simulink library "Lib_Piccolo"  (R2018b)
settings: Solver=VariableStepAuto  StartTime=0.0  StopTime=10.0  RelTol=1e-3
values from neighbouring files (symbols this model uses):
  AccelErrInt2Brakes = 0.15    [SimulationControlConfig16P.m]    (also in SimulationControlConfig16P_LEGACY.m; SimulationControlConfigTAILLESS.m = 0.2; SimulationControlConfigUTAIL.m = 0.2)
  AileronMax = 25    [SimulationControlConfig16P.m]    (also in SimulationControlConfig16P_LEGACY.m; SimulationControlConfigTAILLESS.m; SimulationControlConfigUTAIL.m)
  AileronPower = 0.00268    [SimulationControlConfig16P.m]    (also in SimulationControlConfig16P_LEGACY.m; SimulationControlConfigTAILLESS.m; SimulationControlConfigUTAIL.m)
  AileronSurfaceMax = 45    [SimulationControlConfig16P.m]    (also in SimulationControlConfig16P_LEGACY.m)
  AileronTrim = 0    [SimulationControlConfig16P.m]    (also in SimulationControlConfig16P_LEGACY.m; SimulationControlConfigTAILLESS.m; SimulationControlConfigUTAIL.m)
  Alt = 1000 + TerrainHeight    [SimulationStateConfig.m]
  AltCruise_m = testPlans(testIndx).terrainElevation * 0.3048 + 200    [SimulationControlConfig16P.m]    (also in SimulationControlConfigTAILLESS.m = 1083; SimulationControlConfigUTAIL.m = testPlans(testIndx).terrainElevation * 0.3048 + 152)
  AltitudeRate2PitchCmdIntegratorInit = 0.1    [SimulationControlPre.m]
  AltMax = 10000    [SimulationControlConfig16P.m]    (also in SimulationControlConfig16P_LEGACY.m; SimulationControlConfigTAILLESS.m; SimulationControlConfigUTAIL.m)
  AltMaxAccel = 1.25    [SimulationControlConfig16P.m]    (also in SimulationControlConfig16P_LEGACY.m = 0.9; SimulationControlConfigTAILLESS.m = 1.7; SimulationControlConfigUTAIL.m = 2)
  AltMin = 0    [SimulationControlConfig16P.m]    (also in SimulationControlConfig16P_LEGACY.m; SimulationControlConfigTAILLESS.m; SimulationControlConfigUTAIL.m)
  AltRateCmd2Pitch = 0.50    (= 0.5)    [SimulationControlConfig16P.m]    (also in SimulationControlConfig16P_LEGACY.m = 0.6; SimulationControlConfigTAILLESS.m = 0.2; SimulationControlConfigUTAIL.m = 0.3)
  AltRateError2Pitch = 0.40    (= 0.4)    [SimulationControlConfig16P.m]    (also in SimulationControlConfig16P_LEGACY.m; SimulationControlConfigTAILLESS.m = 0.55; SimulationControlConfigUTAIL.m = 0.55)
  AltRateErrorInt2Pitch = 0.50    (= 0.5)    [SimulationControlConfig16P.m]    (also in SimulationControlConfig16P_LEGACY.m = 0.45; SimulationControlConfigTAILLESS.m; SimulationControlConfigUTAIL.m = 0.75)
  AltRateLpfCutOff = 3    [SimulationControlConfig16P.m]    (also in SimulationControlConfig16P_LEGACY.m; SimulationControlConfigTAILLESS.m = 2; SimulationControlConfigUTAIL.m = 2)
  AutoNosegear2Rudder = 26    [SimulationControlConfig16P.m]    (also in SimulationControlConfig16P_LEGACY.m; SimulationControlConfigTAILLESS.m = 25.2; SimulationControlConfigUTAIL.m = 14)
  b = 5.54    [SimulationControlConfig16P.m]    (also in SimulationControlConfig16P_LEGACY.m; SimulationControlConfigTAILLESS.m = 2.37; SimulationControlConfigUTAIL.m = 2.37)
  Bank2AileronIntegratorInit = 0    [SimulationControlPre.m]
  BankMax_User = BankMax_User/180*pi    (= 0.523598775598)    [SimulationControlConfig16P.m]    (also in SimulationControlConfig16P_LEGACY.m; SimulationControlConfigTAILLESS.m = 0.610865238198; SimulationControlConfigUTAIL.m = 0.628318530718)
  baseLegFlaps = 20    [SimulationControlConfig16P.m]    (also in SimulationControlConfig16P_LEGACY.m = 0; SimulationControlConfigTAILLESS.m = 15; SimulationControlConfigUTAIL.m = 10)
  C = GeneticOpt.C    [SimulationCostFunction.m]
  c = Sw/b    (= 0.841696750903)    [SimulationControlConfig16P.m]    (also in SimulationControlConfig16P_LEGACY.m; SimulationControlConfigTAILLESS.m = 0.354008438819; SimulationControlConfigUTAIL.m = 0.354008438819)
  cell2WheelFactorMG = 5.98    [SimulationSensorConfig16P_LEGACY.m]
  cell2WheelFactorNG = 1    [SimulationSensorConfig16P_LEGACY.m]
  cellSatMaxMG = 15000    [SimulationSensorConfig16P.m]    (also in SimulationSensorConfig16P_LEGACY.m; SimulationSensorConfigTAILLESS7P.m; SimulationSensorConfigUTAIL7P.m)
  cellSatMaxNG = 1000    [SimulationSensorConfig16P.m]    (also in SimulationSensorConfig16P_LEGACY.m; SimulationSensorConfigTAILLESS7P.m; SimulationSensorConfigUTAIL7P.m)
  cellSatMinMG = -15000    [SimulationSensorConfig16P.m]    (also in SimulationSensorConfig16P_LEGACY.m; SimulationSensorConfigTAILLESS7P.m; SimulationSensorConfigUTAIL7P.m)
  cellSatMinNG = -1000    [SimulationSensorConfig16P.m]    (also in SimulationSensorConfig16P_LEGACY.m; SimulationSensorConfigTAILLESS7P.m; SimulationSensorConfigUTAIL7P.m)
  CL_Limit = CL_Max    (= 0.54)    [SimulationControlConfig16P.m]    (also in SimulationControlConfig16P_LEGACY.m; SimulationControlConfigTAILLESS.m; SimulationControlConfigUTAIL.m = 0.53)
  CL_Max = 0.54    [SimulationControlConfig16P.m]    (also in SimulationControlConfig16P_LEGACY.m; SimulationControlConfigTAILLESS.m; SimulationControlConfigUTAIL.m = 0.53)
  CL_Max_Nom = 0.465    [SimulationControlConfig16P.m]    (also in SimulationControlConfig16P_LEGACY.m; SimulationControlConfigTAILLESS.m = 0.39; SimulationControlConfigUTAIL.m)
  CL_Min = 0    [SimulationControlConfig16P.m]    (also in SimulationControlConfig16P_LEGACY.m; SimulationControlConfigTAILLESS.m; SimulationControlConfigUTAIL.m)
  ClimbMaxFraction = 0.35    [SimulationControlConfig16P.m]    (also in SimulationControlConfig16P_LEGACY.m = 0.24; SimulationControlConfigTAILLESS.m = 0.19; SimulationControlConfigUTAIL.m = 0.21)
  ClimboutMaxBank = 7.0    (= 7)    [SimulationControlConfig16P.m]    (also in SimulationControlConfig16P_LEGACY.m; SimulationControlConfigTAILLESS.m = 5; SimulationControlConfigUTAIL.m)
  ClimboutTimer = 7.0    (= 7)    [SimulationControlConfig16P.m]    (also in SimulationControlConfig16P_LEGACY.m; SimulationControlConfigTAILLESS.m; SimulationControlConfigUTAIL.m)
  dCl_per_dFlap = 0.005581818    [SimulationControlConfig16P.m]    (also in SimulationControlConfig16P_LEGACY.m = 0; SimulationControlConfigTAILLESS.m = 0; SimulationControlConfigUTAIL.m = 0)
  DecelerationCmd = 3.1    [SimulationControlConfig16P.m]    (also in SimulationControlConfig16P_LEGACY.m; SimulationControlConfigTAILLESS.m = 0.1; SimulationControlConfigUTAIL.m = 0.1)
  DeRotateLogicEndTimer = abs((NoseDownLimit_Deg-1)/DeRotateRamp_Dps)    [SimulationControlConfig16P.m]    (also in SimulationControlConfig16P_LEGACY.m; SimulationControlConfigTAILLESS.m; SimulationControlConfigUTAIL.m)
  DeRotateLogicHoldNoseUpTimer = 0.1    [SimulationControlConfig16P.m]    (also in SimulationControlConfig16P_LEGACY.m; SimulationControlConfigTAILLESS.m; SimulationControlConfigUTAIL.m)
  DeRotateLogicTimerTimeout = 2    [SimulationControlConfig16P.m]    (also in SimulationControlConfig16P_LEGACY.m; SimulationControlConfigTAILLESS.m; SimulationControlConfigUTAIL.m)
  DeRotateLowerCmdSaturation = 0    [SimulationControlConfig16P.m]    (also in SimulationControlConfig16P_LEGACY.m; SimulationControlConfigTAILLESS.m; SimulationControlConfigUTAIL.m)
  DeRotateRamp_Dps = 3    [SimulationControlConfig16P.m]    (also in SimulationControlConfig16P_LEGACY.m; SimulationControlConfigTAILLESS.m = 8; SimulationControlConfigUTAIL.m = 8)
  DeRotateUpperCmdSaturation = 7    [SimulationControlConfig16P.m]    (also in SimulationControlConfig16P_LEGACY.m; SimulationControlConfigTAILLESS.m; SimulationControlConfigUTAIL.m)
  DescentMaxFraction = 0.22    [SimulationControlConfig16P.m]    (also in SimulationControlConfig16P_LEGACY.m = 0.2; SimulationControlConfigTAILLESS.m = 0.17; SimulationControlConfigUTAIL.m = 0.17)
  DesktopSimTerrainOffset_m = 0.406    [SimulationAircraftConfig.m]
  downwindFlaps = 0    [SimulationControlConfig16P.m]    (also in SimulationControlConfig16P_LEGACY.m; SimulationControlConfigTAILLESS.m; SimulationControlConfigUTAIL.m)
  DP_init = 0.5*1.225*V_init^2    [SimulationControlConfig16P.m]    (also in SimulationControlConfig16P_LEGACY.m; SimulationControlConfigTAILLESS.m; SimulationControlConfigUTAIL.m)
  dscNoiseMG = 1    [SimulationSensorConfig16P_LEGACY.m]
  dscNoiseNG = 0.25    [SimulationSensorConfig16P_LEGACY.m]
  DSCnumBits = 24    [SimulationSensorConfig16P.m]    (also in SimulationSensorConfig16P_LEGACY.m; SimulationSensorConfigTAILLESS7P.m; SimulationSensorConfigUTAIL7P.m)
  DSCRangeMaxMG = 15000    [SimulationSensorConfig16P.m]    (also in SimulationSensorConfig16P_LEGACY.m; SimulationSensorConfigTAILLESS7P.m; SimulationSensorConfigUTAIL7P.m)
  DSCRangeMaxNG = 1000    [SimulationSensorConfig16P.m]    (also in SimulationSensorConfig16P_LEGACY.m; SimulationSensorConfigTAILLESS7P.m; SimulationSensorConfigUTAIL7P.m)
  DSCRangeMinMG = -15000    [SimulationSensorConfig16P.m]    (also in SimulationSensorConfig16P_LEGACY.m; SimulationSensorConfigTAILLESS7P.m; SimulationSensorConfigUTAIL7P.m)
  DSCRangeMinNG = -1000    [SimulationSensorConfig16P.m]    (also in SimulationSensorConfig16P_LEGACY.m; SimulationSensorConfigTAILLESS7P.m; SimulationSensorConfigUTAIL7P.m)
  dt = DLLSim.dt    [SimulationTimeStep.m]    (also in SimulationTrim.m = 0.02)
  EarlyTouchdownThreshold = 3.0    (= 3)    [SimulationControlConfig16P.m]    (also in SimulationControlConfig16P_LEGACY.m; SimulationControlConfigTAILLESS.m = 2.2; SimulationControlConfigUTAIL.m = 2.5)
  ElevatorDeflectionRate = 15    [SimulationControlConfig16P.m]    (also in SimulationControlConfig16P_LEGACY.m = 12; SimulationControlConfigTAILLESS.m = 10; SimulationControlConfigUTAIL.m = 12)
  ElevatorMax = 25    [SimulationControlConfig16P.m]    (also in SimulationControlConfig16P_LEGACY.m; SimulationControlConfigTAILLESS.m; SimulationControlConfigUTAIL.m)
  ElevatorPower = -0.002209    [SimulationControlConfig16P.m]    (also in SimulationControlConfig16P_LEGACY.m; SimulationControlConfigTAILLESS.m = -0.002956; SimulationControlConfigUTAIL.m = -0.00205983)
  ElevatorTrim = -3.5    [SimulationControlConfig16P.m]    (also in SimulationControlConfig16P_LEGACY.m; SimulationControlConfigTAILLESS.m = -6; SimulationControlConfigUTAIL.m = -8)
  elevonBias = 0    [SimulationControlConfig16P.m]    (also in SimulationControlConfig16P_LEGACY.m; SimulationControlConfigTAILLESS.m; SimulationControlConfigUTAIL.m)
  Enable_TAS_Protection = 0    [SimulationControlConfig16P.m]    (also in SimulationControlConfig16P_LEGACY.m; SimulationControlConfigTAILLESS.m; SimulationControlConfigUTAIL.m)
  EnableCrossTrackAbort = 1    [SimulationControlConfig16P.m]    (also in SimulationControlConfigTAILLESS.m; SimulationControlConfigUTAIL.m)
  EnergyBandwidth = 0.02    [SimulationControlConfig16P.m]    (also in SimulationControlConfig16P_LEGACY.m; SimulationControlConfigTAILLESS.m = 0.06; SimulationControlConfigUTAIL.m = 0.06)
  EngineLhFuelCut = 0    [SimulationAircraftConfig.m]
  EngineRhFuelCut = 0    [SimulationAircraftConfig.m]
  FastThrottleRate = 0.075    [SimulationControlConfig16P.m]    (also in SimulationControlConfig16P_LEGACY.m = 0.05; SimulationControlConfigTAILLESS.m = 0.1; SimulationControlConfigUTAIL.m = 0.1)
  FilterWarmUpTime = 2    [SimulationSensorConfig16P.m]    (also in SimulationSensorConfig16P_LEGACY.m; SimulationSensorConfigTAILLESS7P.m; SimulationSensorConfigUTAIL7P.m)
  finalApproachFlaps = 20    [SimulationControlConfig16P.m]    (also in SimulationControlConfig16P_LEGACY.m = 0; SimulationControlConfigTAILLESS.m = 22; SimulationControlConfigUTAIL.m = 10)
  FinalDescentSlope_Deg = testPlans(testIndx).descentSlope    [SimulationControlConfig16P.m]    (also in SimulationControlConfig16P_LEGACY.m; SimulationControlConfigTAILLESS.m; SimulationControlConfigUTAIL.m)
  flapMax = 0    [SimulationControlConfig16P.m]    (also in SimulationControlConfig16P_LEGACY.m; SimulationControlConfigTAILLESS.m; SimulationControlConfigUTAIL.m)
  flapRate = 7.5    [SimulationControlConfig16P.m]    (also in SimulationControlConfig16P_LEGACY.m; SimulationControlConfigTAILLESS.m = 6.6; SimulationControlConfigUTAIL.m)
  FlareHeight = 5    [SimulationControlConfig16P.m]    (also in SimulationControlConfig16P_LEGACY.m = 4.8; SimulationControlConfigTAILLESS.m = 2.5; SimulationControlConfigUTAIL.m = 2)
  FlareVerticalRate_mps = -0.4    [SimulationControlConfig16P.m]    (also in SimulationControlConfig16P_LEGACY.m = -0.5; SimulationControlConfigTAILLESS.m = -0.15; SimulationControlConfigUTAIL.m = -0.15)
  Fp_Aileron = 0.55*2*pi*RollRateLpfCutoff*dt    [SimulationControlConfig16P.m]    (also in SimulationControlConfig16P_LEGACY.m; SimulationControlConfigTAILLESS.m; SimulationControlConfigUTAIL.m)
  Fp_Alt = 0.55*AltBandwidth    (= 0.099)    [SimulationControlConfig16P.m]    (also in SimulationControlConfig16P_LEGACY.m; SimulationControlConfigTAILLESS.m = 0.587477826221; SimulationControlConfigUTAIL.m = 0.69115038379)
  Fp_AltRate = 0.55*2*pi*AltRateLpfCutOff*dt    [SimulationControlConfig16P.m]    (also in SimulationControlConfig16P_LEGACY.m; SimulationControlConfigTAILLESS.m; SimulationControlConfigUTAIL.m)
  Fp_Elevator = 0.55*2*pi*PitchRateLpfCutoff*dt    [SimulationControlConfig16P.m]    (also in SimulationControlConfig16P_LEGACY.m; SimulationControlConfigTAILLESS.m; SimulationControlConfigUTAIL.m)
  Fp_Energy = 0.55*2*pi*EnergyBandwidth    (= 0.069115038379)    [SimulationControlConfig16P.m]    (also in SimulationControlConfig16P_LEGACY.m; SimulationControlConfigTAILLESS.m = 0.207345115137; SimulationControlConfigUTAIL.m = 0.207345115137)
  Fp_Energy2 = 0.55*2*pi*EnergyBandwidth*dt    [SimulationControlConfig16P.m]    (also in SimulationControlConfig16P_LEGACY.m; SimulationControlConfigTAILLESS.m; SimulationControlConfigUTAIL.m)
  Fp_Pitch = 0.55*2*pi*PitchBandwidth    (= 2.76460153516)    [SimulationControlConfig16P.m]    (also in SimulationControlConfig16P_LEGACY.m = 3.11017672705; SimulationControlConfigTAILLESS.m = 3.80132711084; SimulationControlConfigUTAIL.m = 2.41902634326)
  Fp_Pitch_2 = 0.55*2*pi*PitchBandwidth*dt    [SimulationControlConfig16P.m]    (also in SimulationControlConfig16P_LEGACY.m; SimulationControlConfigTAILLESS.m; SimulationControlConfigUTAIL.m)
  Fp_Roll = RollBandwidth^2    (= 1)    [SimulationControlConfig16P.m]    (also in SimulationControlConfig16P_LEGACY.m = 1.44; SimulationControlConfigTAILLESS.m; SimulationControlConfigUTAIL.m)
  Fp_Rudder = 0.55*2*pi*YawRateLpfCutoff*dt    [SimulationControlConfig16P.m]    (also in SimulationControlConfig16P_LEGACY.m; SimulationControlConfigTAILLESS.m; SimulationControlConfigUTAIL.m)
  Fp_TAS = 0.55*2*pi*TASBandwidth    (= 0.103672557568)    [SimulationControlConfig16P.m]    (also in SimulationControlConfig16P_LEGACY.m; SimulationControlConfigTAILLESS.m = 0.172787595947; SimulationControlConfigUTAIL.m = 0.172787595947)
  Fp_TAS_Filter = 2*pi*TasLpfCutoff*dt    [SimulationControlConfig16P.m]    (also in SimulationControlConfig16P_LEGACY.m; SimulationControlConfigTAILLESS.m; SimulationControlConfigUTAIL.m)
  Fp_Turn = 0.55*2*pi*TurnErrLPFcutoff    (= 0.0345575191895)    [SimulationControlConfig16P.m]    (also in SimulationControlConfig16P_LEGACY.m; SimulationControlConfigTAILLESS.m = 0.172787595947; SimulationControlConfigUTAIL.m = 0.172787595947)
  Fp_TurnDerr = 0.55*2*pi*TurnDerivativeLPFcutoff    (= 0.0345575191895)    [SimulationControlConfig16P.m]    (also in SimulationControlConfig16P_LEGACY.m; SimulationControlConfigTAILLESS.m = 0.172787595947; SimulationControlConfigUTAIL.m = 0.172787595947)
  FTV = 3    [SimulationAircraftConfig.m]
  ftvStaticPositionError = 1/1.18    (= 0.847457627119)    [SimulationSensorConfig16P.m]    (also in SimulationSensorConfig16P_LEGACY.m; SimulationSensorConfigTAILLESS7P.m = 1; SimulationSensorConfigUTAIL7P.m = 1)
  g = 9.81    [SimulationStateConfig.m]
  GustSpd_Kts = testPlans(testIndx).gustSpd    [SimulationStateConfig.m]
  GustTriggerVal = testPlans(testIndx).gustTriggerVal    [SimulationStateConfig.m]
  HeadingErr2TurnRate = 0.5    [SimulationControlConfig16P.m]    (also in SimulationControlConfig16P_LEGACY.m; SimulationControlConfigTAILLESS.m; SimulationControlConfigUTAIL.m)
  HeadingErrDer2TurnRate = 0.3    [SimulationControlConfig16P.m]    (also in SimulationControlConfig16P_LEGACY.m; SimulationControlConfigTAILLESS.m; SimulationControlConfigUTAIL.m)
  IASbounce = IASstall*0.8    [SimulationControlPre.m]
  IAScruiseCMD = sqrt(2*m*9.81/(1.225*Sw*CL_cruise))    [SimulationControlConfig16P.m]    (also in SimulationControlConfig16P_LEGACY.m; SimulationControlConfigTAILLESS.m; SimulationControlConfigUTAIL.m)
  IASfinalCMD = 1.12 * IASmin    [SimulationControlConfig16P.m]    (also in SimulationControlConfig16P_LEGACY.m = 1.10 * IASmin; SimulationControlConfigTAILLESS.m = 1.10 * IASmin; SimulationControlConfigUTAIL.m = 1.15 * IASmin)
  IASflareCMD = IASstall    [SimulationControlConfig16P.m]    (also in SimulationControlConfig16P_LEGACY.m; SimulationControlConfigTAILLESS.m; SimulationControlConfigUTAIL.m)
  IASmax = 64    [SimulationControlConfig16P.m]    (also in SimulationControlConfig16P_LEGACY.m = 46; SimulationControlConfigTAILLESS.m = 38.58; SimulationControlConfigUTAIL.m = 35)
  IASmin = sqrt(2*m*9.81/(1.225*Sw*0.9*CL_Max_Nom))    [SimulationControlConfig16P.m]    (also in SimulationControlConfig16P_LEGACY.m; SimulationControlConfigTAILLESS.m; SimulationControlConfigUTAIL.m)
  IASshortCMD = IASstall    [SimulationControlConfig16P.m]    (also in SimulationControlConfig16P_LEGACY.m; SimulationControlConfigTAILLESS.m; SimulationControlConfigUTAIL.m)
  IASstall = sqrt(2*m*9.81/(1.225*Sw*CL_Max))    [SimulationControlConfig16P.m]    (also in SimulationControlConfig16P_LEGACY.m; SimulationControlConfigTAILLESS.m; SimulationControlConfigUTAIL.m)
  inFlight = 1    [SimulationControlConfig16P.m]    (also in SimulationControlConfigTAILLESS.m; SimulationControlConfigUTAIL.m)
  JetCatOffset = 5    [SimulationControlConfig16P.m]    (also in SimulationControlConfig16P_LEGACY.m)
  LaunchRollingElevator = -1.5    [SimulationControlConfig16P.m]    (also in SimulationControlConfig16P_LEGACY.m; SimulationControlConfigTAILLESS.m = 1; SimulationControlConfigUTAIL.m = 1)
  ldg_NosegearMax = 10    [SimulationControlConfig16P.m]    (also in SimulationControlConfig16P_LEGACY.m; SimulationControlConfigTAILLESS.m; SimulationControlConfigUTAIL.m)
  ldg_TrackVyErrInt2Nosegear = 0.1250    (= 0.125)    [SimulationControlConfig16P.m]    (also in SimulationControlConfig16P_LEGACY.m; SimulationControlConfigTAILLESS.m = 0.00714285714286; SimulationControlConfigUTAIL.m = 0.00714285714286)
  ldg_TrackVyErrPro2Nosegear = 0.35    [SimulationControlConfig16P.m]    (also in SimulationControlConfig16P_LEGACY.m; SimulationControlConfigTAILLESS.m = 0.0546666666667; SimulationControlConfigUTAIL.m = 0.0546666666667)
  ldg_TrackY2Vy = 0.07    [SimulationControlConfig16P.m]    (also in SimulationControlConfig16P_LEGACY.m; SimulationControlConfigTAILLESS.m = 0.17; SimulationControlConfigUTAIL.m = 0.17)
  ldg_Vy2NosegearScalingPower = 1.075    [SimulationControlConfig16P.m]    (also in SimulationControlConfig16P_LEGACY.m; SimulationControlConfigTAILLESS.m = 0.6; SimulationControlConfigUTAIL.m = 0.5)
  ldg_Y2VyScalingPower = 0.175    [SimulationControlConfig16P.m]    (also in SimulationControlConfig16P_LEGACY.m; SimulationControlConfigTAILLESS.m = 0; SimulationControlConfigUTAIL.m = 0)
  ldg_YawRate2Nosegear = 0.175    [SimulationControlConfig16P.m]    (also in SimulationControlConfig16P_LEGACY.m; SimulationControlConfigTAILLESS.m = 0.065; SimulationControlConfigUTAIL.m = 0.065)
  LiftSlope = 0.064285    [SimulationControlConfig16P.m]    (also in SimulationControlConfig16P_LEGACY.m; SimulationControlConfigTAILLESS.m = 0.058631; SimulationControlConfigUTAIL.m)
  LPFaileronInit = 0    [SimulationControlPre.m]
  LPFclestInit = 0    [SimulationControlPre.m]
  LPFenergyFFInit = 0    [SimulationControlPre.m]
  LPFtasInit = V_init + 2    [SimulationControlPre.m]
  LPFthrottleInit = ThrottleTrim    [SimulationControlPre.m]
  LPFturnErrInit = 0    [SimulationControlPre.m]
  ... (+115 more)
undefined symbols (not defined in the file or in its folder): abortFlag, alphaHPF, apmDelay, BRWNOUT, CRAWOR, CRAWUR, DiscIntNeverNeededParam, DLLSim, DLLSimStep, ECOMOR, ECOMUR, Fp_Tas, GustTrigger_HeightAgl_m, IPSTAT, LCINTEG, Ldg_Persist_Time, LOWER_FLAGS, MSG_ENABLE, NoiseStd, OLDVAL, OVERRIDE_ENABLE, OVERRIDE_VALUE, REBOOT, reversionEnable, revIASMax, revIASMin, revPitchMax, revPitchMin, revPitchRateMax, revRollMax, revRollRateMax, SAMPLE, SCALON, SensorModel, sigbuilder_block, Sim_Vx, Sim_Vy, Sim_Vz, Sim_Xpos, Sim_Ypos, Sim_Zpos, SYSOR, SYSUR, TARE, TEMPOR, TEMPUR, testIndx, testPlan, testPlans, Trim_piccoloInCmd, Trim_REFSI_FD_IN_nmodeCgShifterCmd_Ft, Trim_REFSI_FD_IN_nmodeFlapLhIBCmd_Deg, Trim_REFSI_FD_IN_nmodeFlapLhOBCmd_Deg, Trim_REFSI_FD_IN_nmodeFlapRhIBCmd_Deg, Trim_REFSI_FD_IN_nmodeFlapRhOBCmd_Deg, Trim_REFSI_FD_IN_nmodeSlatLhCmd_Deg, Trim_REFSI_FD_IN_nmodeSlatRhCmd_Deg, Trim_REFSI_FD_IN_nmodeSplrLhInbdCmd_Deg, Trim_REFSI_FD_IN_nmodeSplrLhOutbdCmd_Deg ... (+5)
libraries: simulink x866, aerolibconvert2 x60, $bdroot x52, aerolibatmos2 x5, dspswit3 x5, simulink_extras x4, dsparch4 x2, Lib_Piccolo_Alt x2, eeGeneralControl x1, dspindex x1
(part 37 of 44)

== system Lib_Piccolo/WOW Archive Container/Load Cell WoW Model 15/Subsystem/Landing Configuration/1-Wheel Timeout ==
  Enable/!Rst : Inport
  Compare To Constant1 : simulink/Logic and Bit Operations/Compare To Constant  relop=>  const=0  OutDataTypeStr=uint8
  Compare To Constant2 : simulink/Logic and Bit Operations/Compare To Constant  relop=>=  const=period  OutDataTypeStr=uint8
  Compare To Constant3 : simulink/Logic and Bit Operations/Compare To Constant  relop===  const=0  OutDataTypeStr=boolean
  Discrete-Time Integrator : DiscreteIntegrator  ExternalReset=level  SampleTime=-1  OutDataTypeStr=double  ICPrevOutput=DiscIntNeverNeededParam  ICPrevScaledInput=DiscIntNeverNeededParam
  Expired : Outport
  wires:
  Compare To Constant3/1 -> Discrete-Time Integrator/2
  Enable/!Rst/1 -> Compare To Constant3/1, Compare To Constant1/1
  Discrete-Time Integrator/1 -> Compare To Constant2/1
  Compare To Constant2/1 -> Expired/1
  Compare To Constant1/1 -> Discrete-Time Integrator/1

== system Lib_Piccolo/WOW Archive Container/Load Cell WoW Model 15/Subsystem/Landing Configuration/Latch ==
  D : Inport
  Enable/!Rst : Inport  Port=2
  AND : Logic  IconShape=distinctive  AllPortsSameDT=off  OutDataTypeStr=boolean
  Constant : Constant
  OR : Logic  Operator=OR  IconShape=distinctive  AllPortsSameDT=off  OutDataTypeStr=boolean
  Switch : Switch  Criteria=u2 > Threshold  Threshold=0.5
  Unit Delay : UnitDelay  SampleTime=-1
  Q_Latched : Outport
  wires:
  Unit Delay/1 -> OR/2
  Switch/1 -> Q_Latched/1, Unit Delay/1
  D/1 -> Switch/3, OR/1
  OR/1 -> AND/1
  AND/1 -> Switch/2
  Enable/!Rst/1 -> AND/2
  Constant/1 -> Switch/1

== system Lib_Piccolo/WOW Archive Container/Load Cell WoW Model 15/Subsystem/Landing Configuration/Persistance Timer ==
  Enable/!Rst : Inport
  Compare To Constant1 : simulink/Logic and Bit Operations/Compare To Constant  relop=>  const=0  OutDataTypeStr=uint8
  Compare To Constant2 : simulink/Logic and Bit Operations/Compare To Constant  relop=>=  const=period  OutDataTypeStr=boolean
  Compare To Constant3 : simulink/Logic and Bit Operations/Compare To Constant  relop===  const=0  OutDataTypeStr=boolean
  Compare To Constant4 : simulink/Logic and Bit Operations/Compare To Constant  relop=>  const=0  OutDataTypeStr=uint8
  Constant : Constant  Value=period
  Discrete-Time Integrator : DiscreteIntegrator  ExternalReset=level  SampleTime=-1  OutDataTypeStr=double  ICPrevOutput=DiscIntNeverNeededParam  ICPrevScaledInput=DiscIntNeverNeededParam
  Switch : Switch  Criteria=u2 > Threshold
  Expired : Outport
  wires:
  Compare To Constant4/1 -> Switch/3
  Constant/1 -> Switch/2
  Switch/1 -> Expired/1
  Compare To Constant3/1 -> Discrete-Time Integrator/2
  Enable/!Rst/1 -> Compare To Constant3/1, Compare To Constant4/1, Compare To Constant1/1
  Discrete-Time Integrator/1 -> Compare To Constant2/1
  Compare To Constant2/1 -> Switch/1
  Compare To Constant1/1 -> Discrete-Time Integrator/1

== system Lib_Piccolo/WOW Archive Container/Load Cell WoW Model 15/Subsystem/Landing Configuration/Primary Latch Timer ==
  Enable/!Rst : Inport
  Compare To Constant1 : simulink/Logic and Bit Operations/Compare To Constant  relop=>  const=0  OutDataTypeStr=uint8
  Compare To Constant2 : simulink/Logic and Bit Operations/Compare To Constant  relop=>=  const=period  OutDataTypeStr=uint8
  Compare To Constant3 : simulink/Logic and Bit Operations/Compare To Constant  relop===  const=0  OutDataTypeStr=boolean
  Discrete-Time Integrator : DiscreteIntegrator  ExternalReset=level  SampleTime=-1  OutDataTypeStr=double  ICPrevOutput=DiscIntNeverNeededParam  ICPrevScaledInput=DiscIntNeverNeededParam
  Expired : Outport
  wires:
  Compare To Constant3/1 -> Discrete-Time Integrator/2
  Enable/!Rst/1 -> Compare To Constant3/1, Compare To Constant1/1
  Discrete-Time Integrator/1 -> Compare To Constant2/1
  Compare To Constant2/1 -> Expired/1
  Compare To Constant1/1 -> Discrete-Time Integrator/1

== system Lib_Piccolo/WOW Archive Container/Load Cell WoW Model 15/Subsystem/T//O Configuration/Latch ==
  D : Inport
  Enable/!Rst : Inport  Port=2
  AND : Logic  IconShape=distinctive  AllPortsSameDT=off  OutDataTypeStr=boolean
  Constant : Constant
  OR : Logic  Operator=OR  IconShape=distinctive  AllPortsSameDT=off  OutDataTypeStr=boolean
  Switch : Switch  Criteria=u2 > Threshold  Threshold=0.5
  Unit Delay : UnitDelay  SampleTime=-1
  Q_Latched : Outport
  wires:
  Constant/1 -> Switch/1
  Enable/!Rst/1 -> AND/2
  AND/1 -> Switch/2
  OR/1 -> AND/1
  D/1 -> OR/1, Switch/3
  Switch/1 -> Unit Delay/1, Q_Latched/1
  Unit Delay/1 -> OR/2

== system Lib_Piccolo/WOW Archive Container/Load Cell WoW Model 15/Subsystem/T//O Configuration/Latch Timer ==
  Enable/!Rst : Inport
  Compare To Constant1 : simulink/Logic and Bit Operations/Compare To Constant  relop=>  const=0  OutDataTypeStr=uint8
  Compare To Constant2 : simulink/Logic and Bit Operations/Compare To Constant  relop=>=  const=period  OutDataTypeStr=uint8
  Compare To Constant3 : simulink/Logic and Bit Operations/Compare To Constant  relop===  const=0  OutDataTypeStr=boolean
  Discrete-Time Integrator : DiscreteIntegrator  ExternalReset=level  SampleTime=-1  OutDataTypeStr=double  ICPrevOutput=DiscIntNeverNeededParam  ICPrevScaledInput=DiscIntNeverNeededParam
  Expired : Outport
  wires:
  Compare To Constant1/1 -> Discrete-Time Integrator/1
  Compare To Constant2/1 -> Expired/1
  Discrete-Time Integrator/1 -> Compare To Constant2/1
  Enable/!Rst/1 -> Compare To Constant1/1, Compare To Constant3/1
  Compare To Constant3/1 -> Discrete-Time Integrator/2

== system Lib_Piccolo/WOW Archive Container/Load Cell WoW Model 15/Subsystem/T//O Configuration/Latch Timer1 ==
  Enable/!Rst : Inport
  Compare To Constant1 : simulink/Logic and Bit Operations/Compare To Constant  relop=>  const=0  OutDataTypeStr=uint8
  Compare To Constant2 : simulink/Logic and Bit Operations/Compare To Constant  relop=>=  const=period  OutDataTypeStr=uint8
  Compare To Constant3 : simulink/Logic and Bit Operations/Compare To Constant  relop===  const=0  OutDataTypeStr=boolean
  Discrete-Time Integrator : DiscreteIntegrator  ExternalReset=level  SampleTime=-1  OutDataTypeStr=double  ICPrevOutput=DiscIntNeverNeededParam  ICPrevScaledInput=DiscIntNeverNeededParam
  Expired : Outport
  wires:
  Compare To Constant3/1 -> Discrete-Time Integrator/2
  Enable/!Rst/1 -> Compare To Constant3/1, Compare To Constant1/1
  Discrete-Time Integrator/1 -> Compare To Constant2/1
  Compare To Constant2/1 -> Expired/1
  Compare To Constant1/1 -> Discrete-Time Integrator/1

== system Lib_Piccolo/WOW Archive Container/Load Cell WoW Model 15/Subsystem/T//O Configuration/Latch Timer2 ==
  Enable/!Rst : Inport
  Compare To Constant1 : simulink/Logic and Bit Operations/Compare To Constant  relop=>  const=0  OutDataTypeStr=uint8
  Compare To Constant2 : simulink/Logic and Bit Operations/Compare To Constant  relop=>=  const=period  OutDataTypeStr=uint8
  Compare To Constant3 : simulink/Logic and Bit Operations/Compare To Constant  relop===  const=0  OutDataTypeStr=boolean
  Discrete-Time Integrator : DiscreteIntegrator  ExternalReset=level  SampleTime=-1  OutDataTypeStr=double  ICPrevOutput=DiscIntNeverNeededParam  ICPrevScaledInput=DiscIntNeverNeededParam
  Expired : Outport
  wires:
  Compare To Constant1/1 -> Discrete-Time Integrator/1
  Compare To Constant2/1 -> Expired/1
  Discrete-Time Integrator/1 -> Compare To Constant2/1
  Enable/!Rst/1 -> Compare To Constant1/1, Compare To Constant3/1
  Compare To Constant3/1 -> Discrete-Time Integrator/2

== system Lib_Piccolo/WOW Archive Container/Load Cell WoW Model 15/Subsystem/T//O Configuration/Latch1 ==
  D : Inport
  Enable/!Rst : Inport  Port=2
  AND : Logic  IconShape=distinctive  AllPortsSameDT=off  OutDataTypeStr=boolean
  Constant : Constant
  OR : Logic  Operator=OR  IconShape=distinctive  AllPortsSameDT=off  OutDataTypeStr=boolean
  Switch : Switch  Criteria=u2 > Threshold  Threshold=0.5
  Unit Delay : UnitDelay  SampleTime=-1
  Q_Latched : Outport
  wires:
  Unit Delay/1 -> OR/2
  Switch/1 -> Q_Latched/1, Unit Delay/1
  D/1 -> Switch/3, OR/1
  OR/1 -> AND/1
  AND/1 -> Switch/2
  Enable/!Rst/1 -> AND/2
  Constant/1 -> Switch/1

== system Lib_Piccolo/WOW Archive Container/Load Cell WoW Model 15/Subsystem/T//O Configuration/Persistance Timer ==
  Enable/!Rst : Inport
  Compare To Constant1 : simulink/Logic and Bit Operations/Compare To Constant  relop=>  const=0  OutDataTypeStr=uint8
  Compare To Constant2 : simulink/Logic and Bit Operations/Compare To Constant  relop=>=  const=period  OutDataTypeStr=boolean
  Compare To Constant3 : simulink/Logic and Bit Operations/Compare To Constant  relop===  const=0  OutDataTypeStr=boolean
  Compare To Constant4 : simulink/Logic and Bit Operations/Compare To Constant  relop=>  const=0  OutDataTypeStr=uint8
  Constant : Constant  Value=period
  Discrete-Time Integrator : DiscreteIntegrator  ExternalReset=level  SampleTime=-1  OutDataTypeStr=double  ICPrevOutput=DiscIntNeverNeededParam  ICPrevScaledInput=DiscIntNeverNeededParam
  Switch : Switch  Criteria=u2 > Threshold
  Expired : Outport
  wires:
  Compare To Constant1/1 -> Discrete-Time Integrator/1
  Compare To Constant2/1 -> Switch/1
  Discrete-Time Integrator/1 -> Compare To Constant2/1
  Enable/!Rst/1 -> Compare To Constant1/1, Compare To Constant4/1, Compare To Constant3/1
  Compare To Constant3/1 -> Discrete-Time Integrator/2
  Switch/1 -> Expired/1
  Constant/1 -> Switch/2
  Compare To Constant4/1 -> Switch/3

== system Lib_Piccolo/WOW Archive Container/Load Cell WoW Model 17/Subsystem/Landing Configuration/1-Wheel Timeout ==
  Enable/!Rst : Inport
  Compare To Constant1 : simulink/Logic and Bit Operations/Compare To Constant  relop=>  const=0  OutDataTypeStr=uint8
  Compare To Constant2 : simulink/Logic and Bit Operations/Compare To Constant  relop=>=  const=period  OutDataTypeStr=uint8
  Compare To Constant3 : simulink/Logic and Bit Operations/Compare To Constant  relop===  const=0  OutDataTypeStr=boolean
  Discrete-Time Integrator : DiscreteIntegrator  ExternalReset=level  SampleTime=-1  OutDataTypeStr=double  ICPrevOutput=DiscIntNeverNeededParam  ICPrevScaledInput=DiscIntNeverNeededParam
  Expired : Outport
  wires:
  Compare To Constant1/1 -> Discrete-Time Integrator/1
  Compare To Constant2/1 -> Expired/1
  Discrete-Time Integrator/1 -> Compare To Constant2/1
  Enable/!Rst/1 -> Compare To Constant1/1, Compare To Constant3/1
  Compare To Constant3/1 -> Discrete-Time Integrator/2

== system Lib_Piccolo/WOW Archive Container/Load Cell WoW Model 17/Subsystem/Landing Configuration/Latch ==
  D : Inport
  Enable/!Rst : Inport  Port=2
  AND : Logic  IconShape=distinctive  AllPortsSameDT=off  OutDataTypeStr=boolean
  Constant : Constant
  OR : Logic  Operator=OR  IconShape=distinctive  AllPortsSameDT=off  OutDataTypeStr=boolean
  Switch : Switch  Criteria=u2 > Threshold  Threshold=0.5
  Unit Delay : UnitDelay  SampleTime=-1
  Q_Latched : Outport
  wires:
  Constant/1 -> Switch/1
  Enable/!Rst/1 -> AND/2
  AND/1 -> Switch/2
  OR/1 -> AND/1
  D/1 -> OR/1, Switch/3
  Switch/1 -> Unit Delay/1, Q_Latched/1
  Unit Delay/1 -> OR/2

== system Lib_Piccolo/WOW Archive Container/Load Cell WoW Model 17/Subsystem/Landing Configuration/Persistance Timer ==
  Enable/!Rst : Inport
  Compare To Constant1 : simulink/Logic and Bit Operations/Compare To Constant  relop=>  const=0  OutDataTypeStr=uint8
  Compare To Constant2 : simulink/Logic and Bit Operations/Compare To Constant  relop=>=  const=period  OutDataTypeStr=boolean
  Compare To Constant3 : simulink/Logic and Bit Operations/Compare To Constant  relop===  const=0  OutDataTypeStr=boolean
  Compare To Constant4 : simulink/Logic and Bit Operations/Compare To Constant  relop=>  const=0  OutDataTypeStr=uint8
  Constant : Constant  Value=period
  Discrete-Time Integrator : DiscreteIntegrator  ExternalReset=level  SampleTime=-1  OutDataTypeStr=double  ICPrevOutput=DiscIntNeverNeededParam  ICPrevScaledInput=DiscIntNeverNeededParam
  Switch : Switch  Criteria=u2 > Threshold
  Expired : Outport
  wires:
  Compare To Constant1/1 -> Discrete-Time Integrator/1
  Compare To Constant2/1 -> Switch/1
  Discrete-Time Integrator/1 -> Compare To Constant2/1
  Enable/!Rst/1 -> Compare To Constant1/1, Compare To Constant4/1, Compare To Constant3/1
  Compare To Constant3/1 -> Discrete-Time Integrator/2
  Switch/1 -> Expired/1
  Constant/1 -> Switch/2
  Compare To Constant4/1 -> Switch/3

== system Lib_Piccolo/WOW Archive Container/Load Cell WoW Model 17/Subsystem/Landing Configuration/Primary Latch Timer ==
  Enable/!Rst : Inport
  Compare To Constant1 : simulink/Logic and Bit Operations/Compare To Constant  relop=>  const=0  OutDataTypeStr=uint8
  Compare To Constant2 : simulink/Logic and Bit Operations/Compare To Constant  relop=>=  const=period  OutDataTypeStr=uint8
  Compare To Constant3 : simulink/Logic and Bit Operations/Compare To Constant  relop===  const=0  OutDataTypeStr=boolean
  Discrete-Time Integrator : DiscreteIntegrator  ExternalReset=level  SampleTime=-1  OutDataTypeStr=double  ICPrevOutput=DiscIntNeverNeededParam  ICPrevScaledInput=DiscIntNeverNeededParam
  Expired : Outport
  wires:
  Compare To Constant1/1 -> Discrete-Time Integrator/1
  Compare To Constant2/1 -> Expired/1
  Discrete-Time Integrator/1 -> Compare To Constant2/1
  Enable/!Rst/1 -> Compare To Constant1/1, Compare To Constant3/1
  Compare To Constant3/1 -> Discrete-Time Integrator/2

== system Lib_Piccolo/WOW Archive Container/Load Cell WoW Model 17/Subsystem/T//O Configuration/Latch ==
  D : Inport
  Enable/!Rst : Inport  Port=2
  AND : Logic  IconShape=distinctive  AllPortsSameDT=off  OutDataTypeStr=boolean
  Constant : Constant
  OR : Logic  Operator=OR  IconShape=distinctive  AllPortsSameDT=off  OutDataTypeStr=boolean
  Switch : Switch  Criteria=u2 > Threshold  Threshold=0.5
  Unit Delay : UnitDelay  SampleTime=-1
  Q_Latched : Outport
  wires:
  Constant/1 -> Switch/1
  Enable/!Rst/1 -> AND/2
  AND/1 -> Switch/2
  OR/1 -> AND/1
  D/1 -> OR/1, Switch/3
  Switch/1 -> Unit Delay/1, Q_Latched/1
  Unit Delay/1 -> OR/2

== system Lib_Piccolo/WOW Archive Container/Load Cell WoW Model 17/Subsystem/T//O Configuration/Latch Timer ==
  Enable/!Rst : Inport
  Compare To Constant1 : simulink/Logic and Bit Operations/Compare To Constant  relop=>  const=0  OutDataTypeStr=uint8
  Compare To Constant2 : simulink/Logic and Bit Operations/Compare To Constant  relop=>=  const=period  OutDataTypeStr=uint8
  Compare To Constant3 : simulink/Logic and Bit Operations/Compare To Constant  relop===  const=0  OutDataTypeStr=boolean
  Discrete-Time Integrator : DiscreteIntegrator  ExternalReset=level  SampleTime=-1  OutDataTypeStr=double  ICPrevOutput=DiscIntNeverNeededParam  ICPrevScaledInput=DiscIntNeverNeededParam
  Expired : Outport
  wires:
  Compare To Constant1/1 -> Discrete-Time Integrator/1
  Compare To Constant2/1 -> Expired/1
  Discrete-Time Integrator/1 -> Compare To Constant2/1
  Enable/!Rst/1 -> Compare To Constant1/1, Compare To Constant3/1
  Compare To Constant3/1 -> Discrete-Time Integrator/2

== system Lib_Piccolo/WOW Archive Container/Load Cell WoW Model 17/Subsystem/T//O Configuration/Latch Timer1 ==
  Enable/!Rst : Inport
  Compare To Constant1 : simulink/Logic and Bit Operations/Compare To Constant  relop=>  const=0  OutDataTypeStr=uint8
  Compare To Constant2 : simulink/Logic and Bit Operations/Compare To Constant  relop=>=  const=period  OutDataTypeStr=uint8
  Compare To Constant3 : simulink/Logic and Bit Operations/Compare To Constant  relop===  const=0  OutDataTypeStr=boolean
  Discrete-Time Integrator : DiscreteIntegrator  ExternalReset=level  SampleTime=-1  OutDataTypeStr=double  ICPrevOutput=DiscIntNeverNeededParam  ICPrevScaledInput=DiscIntNeverNeededParam
  Expired : Outport
  wires:
  Compare To Constant3/1 -> Discrete-Time Integrator/2
  Enable/!Rst/1 -> Compare To Constant3/1, Compare To Constant1/1
  Discrete-Time Integrator/1 -> Compare To Constant2/1
  Compare To Constant2/1 -> Expired/1
  Compare To Constant1/1 -> Discrete-Time Integrator/1

== system Lib_Piccolo/WOW Archive Container/Load Cell WoW Model 17/Subsystem/T//O Configuration/Latch Timer2 ==
  Enable/!Rst : Inport
  Compare To Constant1 : simulink/Logic and Bit Operations/Compare To Constant  relop=>  const=0  OutDataTypeStr=uint8
  Compare To Constant2 : simulink/Logic and Bit Operations/Compare To Constant  relop=>=  const=period  OutDataTypeStr=uint8
  Compare To Constant3 : simulink/Logic and Bit Operations/Compare To Constant  relop===  const=0  OutDataTypeStr=boolean
  Discrete-Time Integrator : DiscreteIntegrator  ExternalReset=level  SampleTime=-1  OutDataTypeStr=double  ICPrevOutput=DiscIntNeverNeededParam  ICPrevScaledInput=DiscIntNeverNeededParam
  Expired : Outport
  wires:
  Compare To Constant1/1 -> Discrete-Time Integrator/1
  Compare To Constant2/1 -> Expired/1
  Discrete-Time Integrator/1 -> Compare To Constant2/1
  Enable/!Rst/1 -> Compare To Constant1/1, Compare To Constant3/1
  Compare To Constant3/1 -> Discrete-Time Integrator/2

== system Lib_Piccolo/WOW Archive Container/Load Cell WoW Model 17/Subsystem/T//O Configuration/Latch1 ==
  D : Inport
  Enable/!Rst : Inport  Port=2
  AND : Logic  IconShape=distinctive  AllPortsSameDT=off  OutDataTypeStr=boolean
  Constant : Constant
  OR : Logic  Operator=OR  IconShape=distinctive  AllPortsSameDT=off  OutDataTypeStr=boolean
  Switch : Switch  Criteria=u2 > Threshold  Threshold=0.5
  Unit Delay : UnitDelay  SampleTime=-1
  Q_Latched : Outport
  wires:
  Unit Delay/1 -> OR/2
  Switch/1 -> Q_Latched/1, Unit Delay/1
  D/1 -> Switch/3, OR/1
  OR/1 -> AND/1
  AND/1 -> Switch/2
  Enable/!Rst/1 -> AND/2
  Constant/1 -> Switch/1

== system Lib_Piccolo/WOW Archive Container/Load Cell WoW Model 17/Subsystem/T//O Configuration/Persistance Timer ==
  Enable/!Rst : Inport
  Compare To Constant1 : simulink/Logic and Bit Operations/Compare To Constant  relop=>  const=0  OutDataTypeStr=uint8
  Compare To Constant2 : simulink/Logic and Bit Operations/Compare To Constant  relop=>=  const=period  OutDataTypeStr=boolean
  Compare To Constant3 : simulink/Logic and Bit Operations/Compare To Constant  relop===  const=0  OutDataTypeStr=boolean
  Compare To Constant4 : simulink/Logic and Bit Operations/Compare To Constant  relop=>  const=0  OutDataTypeStr=uint8
  Constant : Constant  Value=period
  Discrete-Time Integrator : DiscreteIntegrator  ExternalReset=level  SampleTime=-1  OutDataTypeStr=double  ICPrevOutput=DiscIntNeverNeededParam  ICPrevScaledInput=DiscIntNeverNeededParam
  Switch : Switch  Criteria=u2 > Threshold
  Expired : Outport
  wires:
  Compare To Constant1/1 -> Discrete-Time Integrator/1
  Compare To Constant2/1 -> Switch/1
  Discrete-Time Integrator/1 -> Compare To Constant2/1
  Enable/!Rst/1 -> Compare To Constant1/1, Compare To Constant4/1, Compare To Constant3/1
  Compare To Constant3/1 -> Discrete-Time Integrator/2
  Switch/1 -> Expired/1
  Constant/1 -> Switch/2
  Compare To Constant4/1 -> Switch/3

== system Lib_Piccolo/WOW Archive Container/Load Cell WoW Model 2/Subsystem/Landing Configuration/1-Wheel Timeout ==
  Enable/!Rst : Inport
  Compare To Constant1 : simulink/Logic and Bit Operations/Compare To Constant  relop=>  const=0  OutDataTypeStr=uint8
  Compare To Constant2 : simulink/Logic and Bit Operations/Compare To Constant  relop=>=  const=period  OutDataTypeStr=uint8
  Compare To Constant3 : simulink/Logic and Bit Operations/Compare To Constant  relop===  const=0  OutDataTypeStr=boolean
  Discrete-Time Integrator : DiscreteIntegrator  ExternalReset=level  SampleTime=-1  OutDataTypeStr=double  ICPrevOutput=DiscIntNeverNeededParam  ICPrevScaledInput=DiscIntNeverNeededParam
  Expired : Outport
  wires:
  Compare To Constant3/1 -> Discrete-Time Integrator/2
  Enable/!Rst/1 -> Compare To Constant3/1, Compare To Constant1/1
  Discrete-Time Integrator/1 -> Compare To Constant2/1
  Compare To Constant2/1 -> Expired/1
  Compare To Constant1/1 -> Discrete-Time Integrator/1

== system Lib_Piccolo/WOW Archive Container/Load Cell WoW Model 2/Subsystem/Landing Configuration/Latch ==
  D : Inport
  Enable/!Rst : Inport  Port=2
  AND : Logic  IconShape=distinctive  AllPortsSameDT=off  OutDataTypeStr=boolean
  Constant : Constant
  OR : Logic  Operator=OR  IconShape=distinctive  AllPortsSameDT=off  OutDataTypeStr=boolean
  Switch : Switch  Criteria=u2 > Threshold  Threshold=0.5
  Unit Delay : UnitDelay  SampleTime=-1
  Q_Latched : Outport
  wires:
  Unit Delay/1 -> OR/2
  Switch/1 -> Q_Latched/1, Unit Delay/1
  D/1 -> Switch/3, OR/1
  OR/1 -> AND/1
  AND/1 -> Switch/2
  Enable/!Rst/1 -> AND/2
  Constant/1 -> Switch/1

== system Lib_Piccolo/WOW Archive Container/Load Cell WoW Model 2/Subsystem/Landing Configuration/Persistance Timer ==
  Enable/!Rst : Inport
  Compare To Constant1 : simulink/Logic and Bit Operations/Compare To Constant  relop=>  const=0  OutDataTypeStr=uint8
  Compare To Constant2 : simulink/Logic and Bit Operations/Compare To Constant  relop=>=  const=period  OutDataTypeStr=boolean
  Compare To Constant3 : simulink/Logic and Bit Operations/Compare To Constant  relop===  const=0  OutDataTypeStr=boolean
  Compare To Constant4 : simulink/Logic and Bit Operations/Compare To Constant  relop=>  const=0  OutDataTypeStr=uint8
  Constant : Constant  Value=period
  Discrete-Time Integrator : DiscreteIntegrator  ExternalReset=level  SampleTime=-1  OutDataTypeStr=double  ICPrevOutput=DiscIntNeverNeededParam  ICPrevScaledInput=DiscIntNeverNeededParam
  Switch : Switch  Criteria=u2 > Threshold
  Expired : Outport
  wires:
  Compare To Constant4/1 -> Switch/3
  Constant/1 -> Switch/2
  Switch/1 -> Expired/1
  Compare To Constant3/1 -> Discrete-Time Integrator/2
  Enable/!Rst/1 -> Compare To Constant3/1, Compare To Constant4/1, Compare To Constant1/1
  Discrete-Time Integrator/1 -> Compare To Constant2/1
  Compare To Constant2/1 -> Switch/1
  Compare To Constant1/1 -> Discrete-Time Integrator/1

== system Lib_Piccolo/WOW Archive Container/Load Cell WoW Model 2/Subsystem/Landing Configuration/Primary Latch Timer ==
  Enable/!Rst : Inport
  Compare To Constant1 : simulink/Logic and Bit Operations/Compare To Constant  relop=>  const=0  OutDataTypeStr=uint8
  Compare To Constant2 : simulink/Logic and Bit Operations/Compare To Constant  relop=>=  const=period  OutDataTypeStr=uint8
  Compare To Constant3 : simulink/Logic and Bit Operations/Compare To Constant  relop===  const=0  OutDataTypeStr=boolean
  Discrete-Time Integrator : DiscreteIntegrator  ExternalReset=level  SampleTime=-1  OutDataTypeStr=double  ICPrevOutput=DiscIntNeverNeededParam  ICPrevScaledInput=DiscIntNeverNeededParam
  Expired : Outport
  wires:
  Compare To Constant3/1 -> Discrete-Time Integrator/2
  Enable/!Rst/1 -> Compare To Constant3/1, Compare To Constant1/1
  Discrete-Time Integrator/1 -> Compare To Constant2/1
  Compare To Constant2/1 -> Expired/1
  Compare To Constant1/1 -> Discrete-Time Integrator/1

== system Lib_Piccolo/WOW Archive Container/Load Cell WoW Model 2/Subsystem/T//O Configuration/Latch ==
  D : Inport
  Enable/!Rst : Inport  Port=2
  AND : Logic  IconShape=distinctive  AllPortsSameDT=off  OutDataTypeStr=boolean
  Constant : Constant
  OR : Logic  Operator=OR  IconShape=distinctive  AllPortsSameDT=off  OutDataTypeStr=boolean
  Switch : Switch  Criteria=u2 > Threshold  Threshold=0.5
  Unit Delay : UnitDelay  SampleTime=-1
  Q_Latched : Outport
  wires:
  Constant/1 -> Switch/1
  Enable/!Rst/1 -> AND/2
  AND/1 -> Switch/2
  OR/1 -> AND/1
  D/1 -> OR/1, Switch/3
  Switch/1 -> Unit Delay/1, Q_Latched/1
  Unit Delay/1 -> OR/2

== system Lib_Piccolo/WOW Archive Container/Load Cell WoW Model 2/Subsystem/T//O Configuration/Latch Timer ==
  Enable/!Rst : Inport
  Compare To Constant1 : simulink/Logic and Bit Operations/Compare To Constant  relop=>  const=0  OutDataTypeStr=uint8
  Compare To Constant2 : simulink/Logic and Bit Operations/Compare To Constant  relop=>=  const=period  OutDataTypeStr=uint8
  Compare To Constant3 : simulink/Logic and Bit Operations/Compare To Constant  relop===  const=0  OutDataTypeStr=boolean
  Discrete-Time Integrator : DiscreteIntegrator  ExternalReset=level  SampleTime=-1  OutDataTypeStr=double  ICPrevOutput=DiscIntNeverNeededParam  ICPrevScaledInput=DiscIntNeverNeededParam
  Expired : Outport
  wires:
  Compare To Constant1/1 -> Discrete-Time Integrator/1
  Compare To Constant2/1 -> Expired/1
  Discrete-Time Integrator/1 -> Compare To Constant2/1
  Enable/!Rst/1 -> Compare To Constant1/1, Compare To Constant3/1
  Compare To Constant3/1 -> Discrete-Time Integrator/2

== system Lib_Piccolo/WOW Archive Container/Load Cell WoW Model 2/Subsystem/T//O Configuration/Persistance Timer ==
  Enable/!Rst : Inport
  Compare To Constant1 : simulink/Logic and Bit Operations/Compare To Constant  relop=>  const=0  OutDataTypeStr=uint8
  Compare To Constant2 : simulink/Logic and Bit Operations/Compare To Constant  relop=>=  const=period  OutDataTypeStr=uint8
  Compare To Constant3 : simulink/Logic and Bit Operations/Compare To Constant  relop===  const=0  OutDataTypeStr=boolean
  Discrete-Time Integrator : DiscreteIntegrator  ExternalReset=level  SampleTime=-1  OutDataTypeStr=double  ICPrevOutput=DiscIntNeverNeededParam  ICPrevScaledInput=DiscIntNeverNeededParam
  Expired : Outport
  wires:
  Compare To Constant1/1 -> Discrete-Time Integrator/1
  Compare To Constant2/1 -> Expired/1
  Discrete-Time Integrator/1 -> Compare To Constant2/1
  Enable/!Rst/1 -> Compare To Constant1/1, Compare To Constant3/1
  Compare To Constant3/1 -> Discrete-Time Integrator/2

== system Lib_Piccolo/WOW Archive Container/Load Cell WoW Model 3 - LiftOff Delay/Landing Configuration/Latch Timer Selection/Latch Timer Selection ==
  ContactBool : Inport
  AND1 : Logic  Inputs=3  IconShape=distinctive  AllPortsSameDT=off  OutDataTypeStr=boolean
  Constant : Constant  Value=SensorModel.WOW.Cell.useDualTimer
  Invert Contact : simulink/Logic and Bit Operations/Compare To Constant  relop=<  const=0.5  OutDataTypeStr=boolean
  NOT : Logic  Operator=NOT  IconShape=distinctive  AllPortsSameDT=off  OutDataTypeStr=boolean
  Timer Select Latch : Subsystem
  Primary/!Secondary : Outport
  wires:
  NOT/1 -> Primary/!Secondary/1  "Primary/!Secondary"
  ContactBool/1 -> Invert Contact/1
  AND1/1 -> Timer Select Latch/1(D)
  [hasDetected] -> AND1/1
  Invert Contact/1 -> AND1/3
  Timer Select Latch/1(Q_Latched) -> NOT/1  "Seconday/!Primary"
  Constant/1 -> AND1/2
  [apModeEnable] -> Timer Select Latch/2(Enable/!Rst)

== system Lib_Piccolo/WOW Archive Container/Load Cell WoW Model 3 - LiftOff Delay/Landing Configuration/Latch Timer Selection/Primary Latch Timer ==
  Enable/!Rst : Inport
  Compare To Constant1 : simulink/Logic and Bit Operations/Compare To Constant  relop=>  const=0  OutDataTypeStr=uint8
  Compare To Constant2 : simulink/Logic and Bit Operations/Compare To Constant  relop=>=  const=period  OutDataTypeStr=uint8
  Compare To Constant3 : simulink/Logic and Bit Operations/Compare To Constant  relop===  const=0  OutDataTypeStr=boolean
  Discrete-Time Integrator : DiscreteIntegrator  ExternalReset=level  SampleTime=-1  OutDataTypeStr=double  ICPrevOutput=DiscIntNeverNeededParam  ICPrevScaledInput=DiscIntNeverNeededParam
  Expired : Outport
  wires:
  Compare To Constant1/1 -> Discrete-Time Integrator/1
  Compare To Constant2/1 -> Expired/1
  Discrete-Time Integrator/1 -> Compare To Constant2/1
  Enable/!Rst/1 -> Compare To Constant1/1, Compare To Constant3/1
  Compare To Constant3/1 -> Discrete-Time Integrator/2

== system Lib_Piccolo/WOW Archive Container/Load Cell WoW Model 3 - LiftOff Delay/Landing Configuration/Latch Timer Selection/Secondary Latch Timer ==
  Enable/!Rst : Inport
  Compare To Constant2 : simulink/Logic and Bit Operations/Compare To Constant  relop=>=  const=period  OutDataTypeStr=uint8
  Discrete-Time Integrator : DiscreteIntegrator  ExternalReset=level  SampleTime=-1  OutDataTypeStr=double  ICPrevOutput=DiscIntNeverNeededParam  ICPrevScaledInput=DiscIntNeverNeededParam
  NOT1 : Logic  Operator=NOT  IconShape=distinctive  AllPortsSameDT=off  OutDataTypeStr=boolean
  Expired : Outport
  wires:
  Enable/!Rst/1 -> NOT1/1, Discrete-Time Integrator/1
  Compare To Constant2/1 -> Expired/1
  Discrete-Time Integrator/1 -> Compare To Constant2/1  "sTime_s"
  NOT1/1 -> Discrete-Time Integrator/2
